simulink model "HighFrequencyObserver"  (R2026b)
settings: Solver=VariableStepAuto
undefined symbols (not defined in the file or in its folder): hfiCfg, pllCfg, polarityCfg, probeCfg
libraries: AngleTracking x1
settings Model: Creator=24322  LastModifiedBy=24322

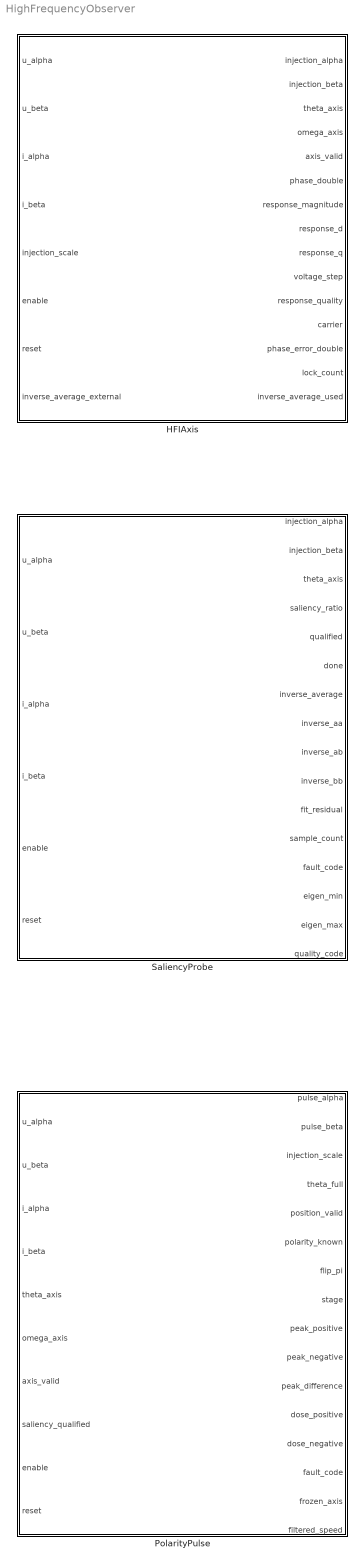
== system HighFrequencyObserver ==
  HFIAxis : Subsystem  mask{cfg=hfiCfg, trackerCfg=pllCfg}
      mask prompts: cfg "HFI axis configuration"; trackerCfg "Doubled phase PLL configuration"
  PolarityPulse : Subsystem  mask{cfg=polarityCfg}
      mask prompts: cfg "Dual pulse polarity configuration"
  SaliencyProbe : Subsystem  mask{cfg=probeCfg}
      mask prompts: cfg "Orthogonal probe configuration"

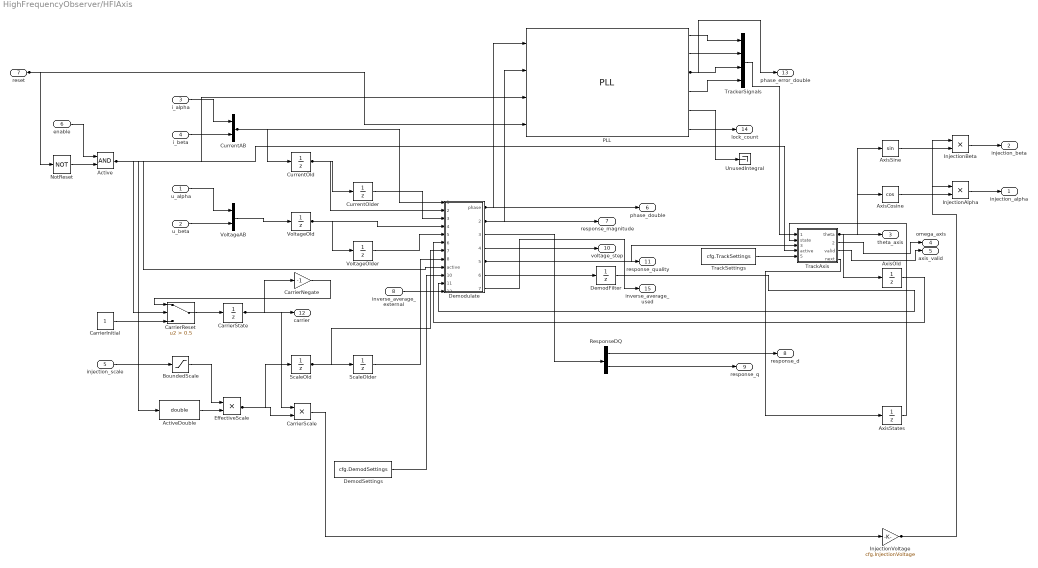
== system HighFrequencyObserver/HFIAxis ==
  u_alpha : Inport  SampleTime=cfg.Ts
  u_beta : Inport  Port=2  SampleTime=cfg.Ts
  i_alpha : Inport  Port=3  SampleTime=cfg.Ts
  i_beta : Inport  Port=4  SampleTime=cfg.Ts
  injection_scale : Inport  Port=5  SampleTime=cfg.Ts
  enable : Inport  Port=6  SampleTime=cfg.Ts
  reset : Inport  Port=7  SampleTime=cfg.Ts
  inverse_average_external : Inport  Port=8  SampleTime=cfg.Ts
  Active : Logic  IconShape=distinctive  AllPortsSameDT=off  OutDataTypeStr=boolean
  ActiveDouble : DataTypeConversion  OutDataTypeStr=double  SaturateOnIntegerOverflow=off  RndMeth=Floor
  AxisCosine : Trigonometry  Operator=cos
  AxisOld : UnitDelay  InitialCondition=cfg.InitialAxis  SampleTime=cfg.Ts
  AxisSine : Trigonometry
  AxisStates : UnitDelay  InitialCondition=cfg.AxisInitialState  SampleTime=cfg.Ts
  BoundedScale : Saturate  UpperLimit=1  LowerLimit=0
  CarrierInitial : Constant
  CarrierNegate : Gain  Gain=-1
  CarrierReset : Switch  Criteria=u2 > Threshold  Threshold=0.5  SaturateOnIntegerOverflow=off  InputSameDT=off
  CarrierScale : Product  Inputs=**
  CarrierState : UnitDelay  InitialCondition=1  SampleTime=cfg.Ts
  CurrentAB : Mux  Inputs=2
  CurrentOld : UnitDelay  InitialCondition=zeros(2,1)  SampleTime=cfg.Ts
  CurrentOlder : UnitDelay  InitialCondition=zeros(2,1)  SampleTime=cfg.Ts
  DemodFilter : UnitDelay  InitialCondition=zeros(2,1)  SampleTime=cfg.Ts
  DemodSettings : Constant  Value=cfg.DemodSettings
  Demodulate : MATLAB Function  TreatAsAtomicUnit=on
  EffectiveScale : Product  Inputs=**
  InjectionAlpha : Product  Inputs=**
  InjectionBeta : Product  Inputs=**
  InjectionVoltage : Gain  Gain=cfg.InjectionVoltage
  NotReset : Logic  Operator=NOT  IconShape=distinctive  AllPortsSameDT=off  OutDataTypeStr=boolean
  PLL : AngleTracking/PLL  pllCfg=trackerCfg
  ResponseDQ : Demux  Outputs=2
  ScaleOld : UnitDelay  SampleTime=cfg.Ts
  ScaleOlder : UnitDelay  SampleTime=cfg.Ts
  TrackAxis : MATLAB Function  TreatAsAtomicUnit=on
  TrackSettings : Constant  Value=cfg.TrackSettings
  TrackerSignals : Mux
  UnusedIntegral : Terminator
  VoltageAB : Mux  Inputs=2
  VoltageOld : UnitDelay  InitialCondition=zeros(2,1)  SampleTime=cfg.Ts
  VoltageOlder : UnitDelay  InitialCondition=zeros(2,1)  SampleTime=cfg.Ts
  injection_alpha : Outport
  injection_beta : Outport  Port=2
  theta_axis : Outport  Port=3
  omega_axis : Outport  Port=4
  axis_valid : Outport  Port=5
  phase_double : Outport  Port=6
  response_magnitude : Outport  Port=7
  response_d : Outport  Port=8
  response_q : Outport  Port=9
  voltage_step : Outport  Port=10
  response_quality : Outport  Port=11
  carrier : Outport  Port=12
  phase_error_double : Outport  Port=13
  lock_count : Outport  Port=14
  inverse_average_used : Outport  Port=15
  wires:
  Demodulate/7(usedAverage) -> inverse_average_used/1
  inverse_average_external/1 -> Demodulate/12(externalAverage)
  Demodulate/5(quality) -> TrackAxis/3(quality), response_quality/1
  Demodulate/4(voltageStep) -> voltage_step/1
  Demodulate/3(responseDQ) -> ResponseDQ/1
  Demodulate/2(magnitude) -> response_magnitude/1, PLL/2
  Demodulate/1(phase) -> phase_double/1, PLL/1
  DemodSettings/1 -> Demodulate/10(settings)
  ScaleOlder/1 -> Demodulate/8(olderScale)
  AxisOld/1 -> Demodulate/6(oldAxis)
  VoltageOlder/1 -> Demodulate/5(olderVoltage)
  CurrentOlder/1 -> Demodulate/3(olderCurrent)
  ScaleOld/1 -> ScaleOlder/1, Demodulate/7(oldScale)
  Active/1 -> PLL/3, CarrierReset/2, ActiveDouble/1, TrackAxis/4(active), Demodulate/9(active)
  CurrentOld/1 -> CurrentOlder/1, Demodulate/2(oldCurrent)
  CurrentAB/1 -> CurrentOld/1, Demodulate/1(current)
  VoltageOld/1 -> VoltageOlder/1, Demodulate/4(oldVoltage)
  Demodulate/6(nextFilter) -> DemodFilter/1
  DemodFilter/1 -> Demodulate/11(filterState)
  u_alpha/1 -> VoltageAB/1
  u_beta/1 -> VoltageAB/2
  i_alpha/1 -> CurrentAB/1
  i_beta/1 -> CurrentAB/2
  VoltageAB/1 -> VoltageOld/1
  reset/1 -> PLL/4, NotReset/1
  NotReset/1 -> Active/2
  enable/1 -> Active/1
  injection_scale/1 -> BoundedScale/1
  BoundedScale/1 -> EffectiveScale/1
  ActiveDouble/1 -> EffectiveScale/2
  EffectiveScale/1 -> CarrierScale/2, ScaleOld/1
  TrackerSignals/1 -> TrackAxis/1(tracker)
  AxisStates/1 -> TrackAxis/2(state)
  TrackSettings/1 -> TrackAxis/5(settings)
  CarrierState/1 -> CarrierScale/1, carrier/1, CarrierNegate/1
  CarrierNegate/1 -> CarrierReset/1
  CarrierInitial/1 -> CarrierReset/3
  CarrierReset/1 -> CarrierState/1
  CarrierScale/1 -> InjectionVoltage/1
  InjectionVoltage/1 -> InjectionBeta/1, InjectionAlpha/1
  AxisCosine/1 -> InjectionAlpha/2
  AxisSine/1 -> InjectionBeta/2
  InjectionAlpha/1 -> injection_alpha/1
  InjectionBeta/1 -> injection_beta/1
  ResponseDQ/1 -> response_d/1
  ResponseDQ/2 -> response_q/1
  PLL/1 -> TrackerSignals/1
  PLL/2 -> TrackerSignals/2
  PLL/3 -> phase_error_double/1, TrackerSignals/3
  PLL/4 -> TrackerSignals/4
  PLL/5 -> UnusedIntegral/1
  PLL/6 -> lock_count/1
  TrackAxis/1(theta) -> theta_axis/1, AxisCosine/1, AxisSine/1, AxisOld/1
  TrackAxis/2(omega) -> omega_axis/1
  TrackAxis/3(valid) -> axis_valid/1
  TrackAxis/4(next) -> AxisStates/1

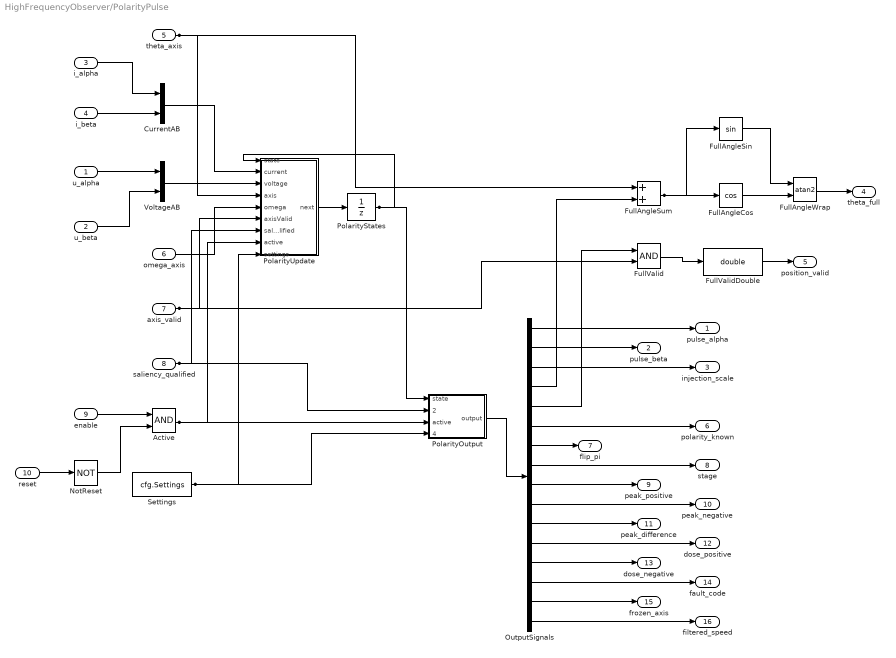
== system HighFrequencyObserver/PolarityPulse ==
  u_alpha : Inport  SampleTime=cfg.Ts
  u_beta : Inport  Port=2  SampleTime=cfg.Ts
  i_alpha : Inport  Port=3  SampleTime=cfg.Ts
  i_beta : Inport  Port=4  SampleTime=cfg.Ts
  theta_axis : Inport  Port=5  SampleTime=cfg.Ts
  omega_axis : Inport  Port=6  SampleTime=cfg.Ts
  axis_valid : Inport  Port=7  SampleTime=cfg.Ts
  saliency_qualified : Inport  Port=8  SampleTime=cfg.Ts
  enable : Inport  Port=9  SampleTime=cfg.Ts
  reset : Inport  Port=10  SampleTime=cfg.Ts
  Active : Logic  IconShape=distinctive  AllPortsSameDT=off  OutDataTypeStr=boolean
  CurrentAB : Mux  Inputs=2
  FullAngleCos : Trigonometry  Operator=cos
  FullAngleSin : Trigonometry
  FullAngleSum : Sum
  FullAngleWrap : Trigonometry  Operator=atan2
  FullValid : Logic  IconShape=distinctive  AllPortsSameDT=off  OutDataTypeStr=boolean
  FullValidDouble : DataTypeConversion  OutDataTypeStr=double  SaturateOnIntegerOverflow=off  RndMeth=Floor
  NotReset : Logic  Operator=NOT  IconShape=distinctive  AllPortsSameDT=off  OutDataTypeStr=boolean
  OutputSignals : Demux  Outputs=16
  PolarityOutput : MATLAB Function  TreatAsAtomicUnit=on
  PolarityStates : UnitDelay  InitialCondition=cfg.InitialState  SampleTime=cfg.Ts
  PolarityUpdate : MATLAB Function  TreatAsAtomicUnit=on
  Settings : Constant  Value=cfg.Settings
  VoltageAB : Mux  Inputs=2
  pulse_alpha : Outport
  pulse_beta : Outport  Port=2
  injection_scale : Outport  Port=3
  theta_full : Outport  Port=4
  position_valid : Outport  Port=5
  polarity_known : Outport  Port=6
  flip_pi : Outport  Port=7
  stage : Outport  Port=8
  peak_positive : Outport  Port=9
  peak_negative : Outport  Port=10
  peak_difference : Outport  Port=11
  dose_positive : Outport  Port=12
  dose_negative : Outport  Port=13
  fault_code : Outport  Port=14
  frozen_axis : Outport  Port=15
  filtered_speed : Outport  Port=16
  wires:
  OutputSignals/16 -> filtered_speed/1
  OutputSignals/15 -> frozen_axis/1
  OutputSignals/14 -> fault_code/1
  OutputSignals/13 -> dose_negative/1
  OutputSignals/12 -> dose_positive/1
  OutputSignals/11 -> peak_difference/1
  OutputSignals/10 -> peak_negative/1
  OutputSignals/9 -> peak_positive/1
  OutputSignals/8 -> stage/1
  OutputSignals/7 -> flip_pi/1
  OutputSignals/6 -> polarity_known/1
  OutputSignals/3 -> injection_scale/1
  OutputSignals/2 -> pulse_beta/1
  OutputSignals/1 -> pulse_alpha/1
  OutputSignals/5 -> FullValid/1
  OutputSignals/4 -> FullAngleSum/2
  FullValidDouble/1 -> position_valid/1
  FullAngleWrap/1 -> theta_full/1
  FullValid/1 -> FullValidDouble/1
  FullAngleCos/1 -> FullAngleWrap/2
  FullAngleSin/1 -> FullAngleWrap/1
  FullAngleSum/1 -> FullAngleSin/1, FullAngleCos/1
  PolarityOutput/1(output) -> OutputSignals/1
  PolarityUpdate/1(next) -> PolarityStates/1
  Settings/1 -> PolarityUpdate/9(settings), PolarityOutput/4(settings)
  Active/1 -> PolarityUpdate/8(active), PolarityOutput/3(active)
  saliency_qualified/1 -> PolarityUpdate/7(saliencyQualified), PolarityOutput/2(saliencyQualified)
  axis_valid/1 -> FullValid/2, PolarityUpdate/6(axisValid)
  omega_axis/1 -> PolarityUpdate/5(omega)
  theta_axis/1 -> FullAngleSum/1, PolarityUpdate/4(axis)
  VoltageAB/1 -> PolarityUpdate/3(voltage)
  CurrentAB/1 -> PolarityUpdate/2(current)
  PolarityStates/1 -> PolarityUpdate/1(state), PolarityOutput/1(state)
  enable/1 -> Active/1
  NotReset/1 -> Active/2
  reset/1 -> NotReset/1
  i_beta/1 -> CurrentAB/2
  i_alpha/1 -> CurrentAB/1
  u_beta/1 -> VoltageAB/2
  u_alpha/1 -> VoltageAB/1

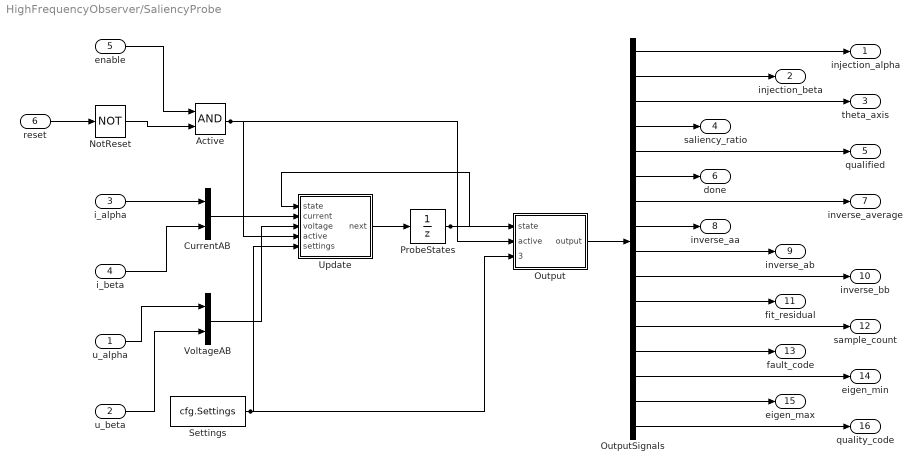
== system HighFrequencyObserver/SaliencyProbe ==
  u_alpha : Inport  SampleTime=cfg.Ts
  u_beta : Inport  Port=2  SampleTime=cfg.Ts
  i_alpha : Inport  Port=3  SampleTime=cfg.Ts
  i_beta : Inport  Port=4  SampleTime=cfg.Ts
  enable : Inport  Port=5  SampleTime=cfg.Ts
  reset : Inport  Port=6  SampleTime=cfg.Ts
  Active : Logic  IconShape=distinctive  AllPortsSameDT=off  OutDataTypeStr=boolean
  CurrentAB : Mux  Inputs=2
  NotReset : Logic  Operator=NOT  IconShape=distinctive  AllPortsSameDT=off  OutDataTypeStr=boolean
  Output : MATLAB Function  TreatAsAtomicUnit=on
  OutputSignals : Demux  Outputs=16
  ProbeStates : UnitDelay  InitialCondition=cfg.InitialState  SampleTime=cfg.Ts
  Settings : Constant  Value=cfg.Settings
  Update : MATLAB Function  TreatAsAtomicUnit=on
  VoltageAB : Mux  Inputs=2
  injection_alpha : Outport
  injection_beta : Outport  Port=2
  theta_axis : Outport  Port=3
  saliency_ratio : Outport  Port=4
  qualified : Outport  Port=5
  done : Outport  Port=6
  inverse_average : Outport  Port=7
  inverse_aa : Outport  Port=8
  inverse_ab : Outport  Port=9
  inverse_bb : Outport  Port=10
  fit_residual : Outport  Port=11
  sample_count : Outport  Port=12
  fault_code : Outport  Port=13
  eigen_min : Outport  Port=14
  eigen_max : Outport  Port=15
  quality_code : Outport  Port=16
  wires:
  OutputSignals/16 -> quality_code/1
  OutputSignals/15 -> eigen_max/1
  OutputSignals/14 -> eigen_min/1
  OutputSignals/13 -> fault_code/1
  OutputSignals/12 -> sample_count/1
  OutputSignals/11 -> fit_residual/1
  OutputSignals/10 -> inverse_bb/1
  OutputSignals/9 -> inverse_ab/1
  OutputSignals/8 -> inverse_aa/1
  OutputSignals/7 -> inverse_average/1
  OutputSignals/6 -> done/1
  OutputSignals/5 -> qualified/1
  OutputSignals/4 -> saliency_ratio/1
  OutputSignals/3 -> theta_axis/1
  OutputSignals/2 -> injection_beta/1
  OutputSignals/1 -> injection_alpha/1
  Output/1(output) -> OutputSignals/1
  Update/1(next) -> ProbeStates/1
  Settings/1 -> Update/5(settings), Output/3(settings)
  Active/1 -> Update/4(active), Output/2(active)
  VoltageAB/1 -> Update/3(voltage)
  CurrentAB/1 -> Update/2(current)
  ProbeStates/1 -> Update/1(state), Output/1(state)
  enable/1 -> Active/1
  NotReset/1 -> Active/2
  reset/1 -> NotReset/1
  i_beta/1 -> CurrentAB/2
  i_alpha/1 -> CurrentAB/1
  u_beta/1 -> VoltageAB/2
  u_alpha/1 -> VoltageAB/1

== matlab function HighFrequencyObserver/HFIAxis/TrackAxis ==
  data: tracker input; theta output; state input; quality input; active input; settings input; omega output; valid output; next output
function [theta,omega,valid,next]=hfi_track_axis(tracker,state,quality,active,settings)
%HFI_TRACK_AXIS Unwrap doubled PLL phase without introducing pi jumps.
% tracker=[theta_double;omega_double;phase_error_double;pll_valid].
% state=[last_continuous_axis;last_tracker_phase]. No polarity is identified.
% settings=[initial_axis;initial_tracker_phase;max_electrical_speed].
%#codegen
theta=settings(1);omega=zeros(1,'like',state);valid=zeros(1,'like',state);
next=[settings(1);settings(2)];
if ~active,return;end
delta=0.5*atan2(sin(tracker(1)-state(2)),cos(tracker(1)-state(2)));
theta=atan2(sin(state(1)+delta),cos(state(1)+delta));
omega=0.5*tracker(2);next=[theta;tracker(1)];
valid=cast(tracker(4)>0.5 && quality>0.5 && abs(omega)<=settings(3),'like',state);
end

== matlab function HighFrequencyObserver/HFIAxis/Demodulate ==
  data: current input; phase output; oldCurrent input; olderCurrent input; oldVoltage input; olderVoltage input; oldAxis input; oldScale input; olderScale input; active input; settings input; magnitude output; responseDQ output; voltageStep output; quality output; filterState input; nextFilter output; externalAverage input; usedAverage output
function [phase,magnitude,responseDQ,voltageStep,quality,nextFilter,usedAverage]=hfi_demodulate(current,oldCurrent,olderCurrent,oldVoltage,olderVoltage,oldAxis,oldScale,olderScale,active,settings,filterState,externalAverage)
%HFI_DEMODULATE Two-interval demodulation with measured applied voltages.
% current[k] closes interval u[k-1]; u[k] must NOT feed this calculation.
% settings=[Ts;Vh;inverse_average;cross_phase;min_voltage_step;max_cross_fraction;min_response;max_response;min_scale;filter_a;use_external_average].
%#codegen
phase=zeros(1,'like',current);magnitude=zeros(1,'like',current);
responseDQ=zeros(2,1,'like',current);voltageStep=zeros(1,'like',current);quality=zeros(1,'like',current);
nextFilter=zeros(2,1,'like',current);
usedAverage=zeros(1,'like',current);
if ~active || ~all(isfinite([current;oldCurrent;olderCurrent;oldVoltage;olderVoltage;oldAxis;oldScale;olderScale;filterState]))
    return;
end
if oldScale<settings(9) || olderScale<settings(9),return;end
cosine=cos(oldAxis);sine=sin(oldAxis);deltaVoltage=oldVoltage-olderVoltage;
projection=cosine*deltaVoltage(1)+sine*deltaVoltage(2);
cross=-sine*deltaVoltage(1)+cosine*deltaVoltage(2);
voltageStep=projection;
if abs(projection)<settings(5) || abs(cross)>settings(6)*abs(projection),return;end
average=settings(3);
if settings(11)>0.5
    if ~isfinite(externalAverage) || externalAverage<=0,return;end
    average=externalAverage;
end
usedAverage=average;
secondDifference=current-2*oldCurrent+olderCurrent;
response=secondDifference/(settings(1)*projection);
responseDQ=[cosine*response(1)+sine*response(2);-sine*response(1)+cosine*response(2)];
saliency=[responseDQ(1)-average;responseDQ(2)];
rotation=2*oldAxis-settings(4);rotationCos=cos(rotation);rotationSin=sin(rotation);
stationary=[rotationCos*saliency(1)-rotationSin*saliency(2);rotationSin*saliency(1)+rotationCos*saliency(2)];
nextFilter=settings(10)*filterState+(1-settings(10))*stationary;
phase=atan2(nextFilter(2),nextFilter(1));
magnitude=hypot(nextFilter(1),nextFilter(2))*settings(1)*abs(projection)/2;
quality=cast(magnitude>=settings(7) && magnitude<=settings(8),'like',current);
if quality<0.5,magnitude(:)=0;end
end

== matlab function HighFrequencyObserver/SaliencyProbe/Update ==
  data: state input; next output; current input; voltage input; active input; settings input
function next=hfi_probe_update(state,current,voltage,active,settings)
%HFI_PROBE_UPDATE Fit actual interval voltage changes to second current changes.
% state=[tick,count,i1(2),i2(2),u1(2),u2(2),XX11,XX12,XX22,YX(4),YY,fault].
% i[k] closes u[k-1]; current applied u[k] is stored ONLY for the next sample.
% The completed snapshot is held until disable/reset, not a running protection.
%#codegen
next=state;
if ~active,next(:)=0;return;end
total=settings(3)+settings(4);
if state(1)>=total || state(19)>0,return;end
if ~all(isfinite([current;voltage]))
    next(19)=2;return;
end
if hypot(current(1),current(2))>settings(12)
    next(19)=1;return;
end
if state(1)>=settings(3)
    x=state(7:8)-state(9:10);
    y=(current-2*state(3:4)+state(5:6))/settings(1);
    next(2)=state(2)+1;
    next(11)=state(11)+x(1)*x(1);next(12)=state(12)+x(1)*x(2);next(13)=state(13)+x(2)*x(2);
    next(14)=state(14)+y(1)*x(1);next(15)=state(15)+y(1)*x(2);
    next(16)=state(16)+y(2)*x(1);next(17)=state(17)+y(2)*x(2);
    next(18)=state(18)+dot(y,y);
end
next(1)=state(1)+1;
next(5:6)=state(3:4);next(3:4)=current;
next(9:10)=state(7:8);next(7:8)=voltage;
end

== matlab function HighFrequencyObserver/SaliencyProbe/Output ==
  data: state input; output output; active input; settings input
function output=hfi_probe_output(state,active,settings)
%HFI_PROBE_OUTPUT Causal excitation plus measured-tensor qualification.
% outputs=[requestAB(2),axis,ratio,qualified,done,inverseAverage,tensor(3),residual,count,fault,eigenMin,eigenMax,qualityCode].
% qualityCode:0 collecting,1 qualified,2 weak voltage,3 eigen range,4 saliency,
%             5 fit residual,6 asymmetry,7 input/current fault.
%#codegen
output=zeros(16,1,'like',state);
if ~active,return;end
done=state(1)>=settings(3)+settings(4) || state(19)>0;
output(6)=cast(done,'like',state);output(12)=state(2);output(13)=state(19);
if state(19)>0,output(16)=7;return;end
if ~done
    phase=mod(state(1),4);axis=settings(13);amplitude=settings(2);
    if phase>=2,axis=axis+pi/2;end
    if mod(phase,2)==1,amplitude=-amplitude;end
    output(1:2)=amplitude*[cos(axis);sin(axis)];
end
if state(2)<4,return;end
xx11=state(11);xx12=state(12);xx22=state(13);determinant=xx11*xx22-xx12*xx12;
if determinant<=0
    if done,output(16)=2;end
    return;
end
a11=(state(14)*xx22-state(15)*xx12)/determinant;
a12=(state(15)*xx11-state(14)*xx12)/determinant;
a21=(state(16)*xx22-state(17)*xx12)/determinant;
a22=(state(17)*xx11-state(16)*xx12)/determinant;
cross=0.5*(a12+a21);average=0.5*(a11+a22);
radius=hypot(0.5*(a11-a22),cross);eigenMin=average-radius;eigenMax=average+radius;
ratio=radius/max(abs(average),eps);
angle=0.5*atan2(2*cross,a11-a22)-0.5*settings(14);
residualEnergy=max(state(18)-(a11*state(14)+a12*state(15)+a21*state(16)+a22*state(17)),0);
residual=sqrt(residualEnergy/max(state(18),eps));
asymmetry=sqrt(2)*abs(a12-a21)/max(abs(a11+a22),eps);
voltageMinEigen=0.5*(xx11+xx22)-hypot(0.5*(xx11-xx22),xx12);
voltageRms=sqrt(max(voltageMinEigen,0)/state(2));
output(3)=atan2(sin(angle),cos(angle));output(4)=ratio;output(7)=average;
output(8:10)=[a11;cross;a22];output(11)=residual;output(14:15)=[eigenMin;eigenMax];
if ~done,return;end
code=1;
if voltageRms<settings(11),code=2;
elseif eigenMin<settings(7) || eigenMax>settings(8),code=3;
elseif ratio<settings(5) || ratio>settings(6),code=4;
elseif residual>settings(9),code=5;
elseif asymmetry>settings(10),code=6;
end
output(16)=code;output(5)=cast(code==1,'like',state);
end

== matlab function HighFrequencyObserver/PolarityPulse/PolarityUpdate ==
  data: state input; next output; current input; voltage input; axis input; omega input; axisValid input; saliencyQualified input; active input; settings input
function next=hfi_polarity_update(state,current,voltage,axis,omega,axisValid,saliencyQualified,active,settings)
%HFI_POLARITY_UPDATE Stop HFI, apply equal dual pulses and compare decay peaks.
% state=[stage,ticks,total,axisCount,decayCount,frozenAxis,peakP,peakN,doseP,
%        doseN,crossDose,baselineP,baselineN,flip,known,fault,speedLP,uOld(2)].
% stages0init1wait2settle3positive4decay5negative6decay7track8fault.
% Current[k] closes stored actual voltage[k-1], including execution delay.
%#codegen
next=state;
if ~active,next(:)=0;return;end
stage=state(1);
if stage==8,return;end
if ~all(isfinite([current;voltage;axis;omega;axisValid;saliencyQualified]))
    next(1)=8;next(16)=7;return;
end
if stage<7 && hypot(current(1),current(2))>settings(11)
    next(1)=8;next(16)=1;return;
end
next(17)=settings(19)*state(17)+(1-settings(19))*omega;
next(18:19)=voltage;
if stage>=2 && saliencyQualified<.5,next(1)=8;next(16)=6;return;end
if stage==7,return;end
next(3)=state(3)+1;next(2)=state(2)+1;
if stage==0,next(1)=1;next(2)=0;return;end
if next(3)>settings(9),next(1)=8;next(16)=8;return;end
cosine=cos(state(6));sine=sin(state(6));id=cosine*current(1)+sine*current(2);
u=cosine*state(18)+sine*state(19);uq=-sine*state(18)+cosine*state(19);
if stage==3 || stage==4
    next(7)=max(state(7),id-state(12));
    if abs(u)>=settings(18)
        if u<0,next(1)=8;next(16)=4;return;end
        next(9)=state(9)+settings(1)*u;next(11)=state(11)+settings(1)*abs(uq);
    end
elseif stage==5 || stage==6
    next(8)=max(state(8),state(13)-id);
    if abs(u)>=settings(18)
        if u>0,next(1)=8;next(16)=4;return;end
        next(10)=state(10)-settings(1)*u;next(11)=state(11)+settings(1)*abs(uq);
    end
end
switch stage
    case 1
        good=axisValid>.5 && saliencyQualified>.5 && abs(next(17))<=settings(12);
        if good,next(4)=state(4)+1;else,next(4)=0;end
        if next(4)>=settings(4)
            next(1)=2;next(2)=0;next(5)=0;next(6)=axis;
        elseif next(2)>=settings(7),next(1)=8;next(16)=2;
        end
    case {2,4,6}
        if hypot(current(1),current(2))<=settings(10),next(5)=state(5)+1;else,next(5)=0;end
        if next(2)>=settings(5) && next(5)>=settings(6)
            next(2)=0;next(5)=0;
            if stage==2,next(1)=3;next(12)=id;
            elseif stage==4,next(1)=5;next(13)=id;
            else
                meanDose=.5*(next(9)+next(10));mismatch=abs(next(9)-next(10))/max(meanDose,eps);
                crossFraction=next(11)/max(next(9)+next(10),eps);
                difference=next(7)-next(8);relative=abs(difference)/max(.5*(next(7)+next(8)),eps);
                if min(next(9),next(10))<settings(15) || mismatch>settings(16) || crossFraction>settings(17)
                    next(1)=8;next(16)=4;
                elseif abs(difference)<settings(13) || relative<settings(14)
                    next(1)=8;next(16)=5;
                else
                    next(1)=7;next(14)=cast(difference<0,'like',state);next(15)=1;
                end
            end
        elseif next(2)>=settings(8),next(1)=8;next(16)=3;
        end
    case {3,5}
        if next(2)>=settings(3),next(1)=stage+1;next(2)=0;next(5)=0;end
end
end

== matlab function HighFrequencyObserver/PolarityPulse/PolarityOutput ==
  data: state input; output output; saliencyQualified input; active input; settings input
function output=hfi_polarity_output(state,saliencyQualified,active,settings)
%HFI_POLARITY_OUTPUT State-only requests; external wrap/validity use HFI lock.
% [pulseAB(2),hfiScale,thetaOffset,ready,known,flip,stage,peaks(2),difference,
%  doses(2),fault,frozenAxis,speedLP]. Positive d saturation lowers Ld.
%#codegen
output=zeros(16,1,'like',state);
if ~active || ~isfinite(saliencyQualified),return;end
stage=state(1);if stage==0,stage=1;end
if (stage==1 || stage==7) && saliencyQualified>.5,output(3)=1;end
amplitude=zeros(1,'like',state);
if stage==3,amplitude=settings(2);elseif stage==5,amplitude=-settings(2);end
output(1:2)=amplitude*[cos(state(6));sin(state(6))];
output(4)=pi*state(14);
output(5)=cast(stage==7 && state(15)>.5 && saliencyQualified>.5,'like',state);
output(6)=state(15);output(7)=state(14);output(8)=stage;
output(9:10)=state(7:8);output(11)=state(7)-state(8);output(12:13)=state(9:10);
output(14)=state(16);output(15)=state(6);output(16)=state(17);
end
